simulink model "DC_motor_model"  (R2025b)
settings: Solver=VariableStepAuto  StartTime=0.0  StopTime=10.0  RelTol=1e-3
values from neighbouring files (symbols this model uses):
  K_i = 7.31220718673    [motorbike_cruise_control.mat]
  K_p = 0.333562341287    [motorbike_cruise_control.mat]
  V_max = 11.53    [motorbike_cruise_control.mat]
undefined symbols (not defined in the file or in its folder): K_d, T_s
libraries: slpidlib x1
settings Model: Creator=konstantinos  LastModifiedBy=konstantinos

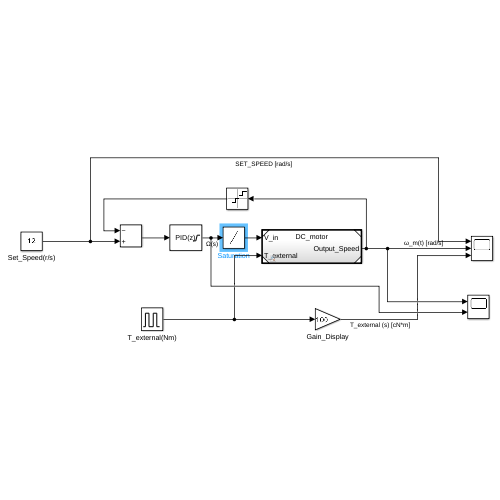
[thumbnail: Simulink's stored preview of the top-level diagram]
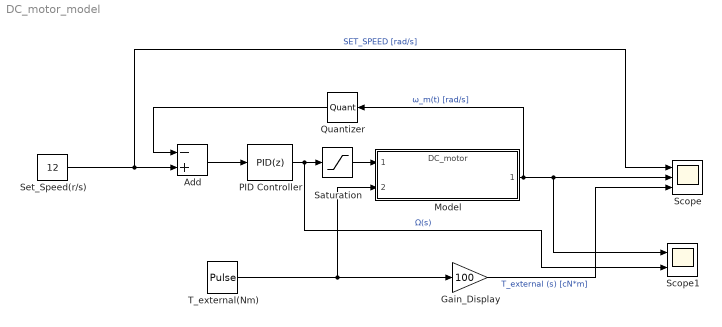
== system DC_motor_model ==
  Add : Sum  Inputs=-+
  Gain_Display : Gain  Gain=100
  Model : ModelReference  ModelNameDialog=DC_motor.slx  SimulationMode=Normal  ModelReferenceVersion=1.4
  PID Controller : slpidlib/PID Controller  Controller=PID  Form=Parallel  TimeDomain=Discrete-time  UseExternalTs=off  SampleTime=T_s  IntegratorMethod=Trapezoidal  FilterMethod=Trapezoidal  ControllerParametersSource=internal  P=K_p  I=K_i  UseKiTs=off  D=K_d  UseExternalDerivativeSource=off  N=100  UseFilter=on  TunerSelectOption=Transfer Function Based (PID Tuner App)  InitialConditionSource=internal  InitialConditionForIntegrator=0  InitialConditionForFilter=0  DifferentiatorICPrevScaledInput=0  ExternalReset=none  TrackingMode=off  Kt=1  LimitOutput=on  SatLimitsSource=internal  UpperSaturationLimit=11.1  LowerSaturationLimit=-11.1  LinearizeAsGain=on  AntiWindupMode=back-calculation  Kb=1  LimitIntegrator=off  UpperIntegratorSaturationLimit=inf  LowerIntegratorSaturationLimit=-inf  POutMin=[]  POutMax=[]  IOutMin=[]  IOutMax=[]  DOutMin=[]  DOutMax=[]  NOutMin=[]  NOutMax=[]  SumOutMin=[]  SumOutMax=[]  SaturationOutMin=[]  SaturationOutMax=[]  PParamMin=[]  PParamMax=[]  IParamMin=[]  IParamMax=[]  DParamMin=[]  DParamMax=[]  NParamMin=[]  NParamMax=[]  KbParamMin=[]  KbParamMax=[]  KtParamMin=[]  KtParamMax=[]  KbOutMin=[]  KbOutMax=[]  KtOutMin=[]  KtOutMax=[]  IntegratorOutMin=[]  IntegratorOutMax=[]  FilterOutMin=[]  FilterOutMax=[]  SumI1OutMin=[]  SumI1OutMax=[]  SumI2OutMin=[]  SumI2OutMax=[]  SumI3OutMin=[]  SumI3OutMax=[]  SumI4OutMin=[]  SumI4OutMax=[]  SumDOutMin=[]  SumDOutMax=[]  DifferentiatorOutMin=[]  DifferentiatorOutMax=[]  FilterDiffOutCoefMin=[]  FilterDiffOutCoefMax=[]  ReciprocalOutMin=[]  ReciprocalOutMax=[]  SumDenOutMin=[]  SumDenOutMax=[]  SumNumOutMin=[]  SumNumOutMax=[]  DivideOutMin=[]  DivideOutMax=[]  UdiffTsProdOutMin=[]  UdiffTsProdOutMax=[]  NTsProdOutMin=[]  NTsProdOutMax=[]  UintegralTsProdOutMin=[]  UintegralTsProdOutMax=[]  UngainTsProdOutMin=[]  UngainTsProdOutMax=[]  ClampingZeroOutDataTypeStr=Inherit: Inherit via back propagation  ClampingZeroOutMin=[]  ClampingZeroOutMax=[]  FilterDenConstantOutDataTypeStr=Inherit: Inherit via back propagation  FilterDenConstantOutMin=[]  FilterDenConstantOutMax=[]  PCopyOutDataTypeStr=Inherit: Inherit via back propagation  PCopyOutMin=[]  PCopyOutMax=[]  NCopyOutDataTypeStr=Inherit: Inherit via back propagation  NCopyOutMin=[]  NCopyOutMax=[]  IntegratorContinuousStateAttributes=''  IntegratorStateMustResolveToSignalObject=off  IntegratorRTWStateStorageClass=Auto  FilterContinuousStateAttributes=''  FilterStateMustResolveToSignalObject=off  FilterRTWStateStorageClass=Auto  ParallelPVariant=InternalParameters  IdealPVariant=Disabled  IVariant=InternalParameters  DVariant=InternalParameters  IntegratorVariant=Discrete  SatVariant=Enabled  AWVariant=BackCalculation  PCopyVariant=Disabled  TRVariant=Disabled  FdbkBlocksVariant=Feedback  IdealPFdbkVariant=Passthrough  SatFdbkVariant=Enabled  DerivativeFilterVariant=TrapezoidalFilter  NVariant=InternalParameters  NCopyVariant=InternalParameters  FilterICVariant=InternalICsFilter  IntegratorICVariant=InternalICs  ExternalResetVariant=Disabled  TRSumVariant=Passthrough  SumFdbkVariant=Enabled  SumVariant=Sum_PID  TsampFilterVariant=InternalTs  TsampNgainVariant=Passthrough  TsampIntegralVariant=Disabled_SignalSpec  ExternalSaturationOutDataTypeStr=Inherit: Same as second input  DerivativeSourceVariant=ErrorSignal  PreIntVariant=InternalPreInt
  Quantizer : Quantizer  QuantizationInterval=2*pi/1200
  Saturation : Saturate  UpperLimit=V_max  LowerLimit=-V_max
  Scope : Scope  NumInputPorts=3
      settings: ActiveDisplayYMinimum=-9.4133876300961674  ActiveDisplayYMaximum=29.145633273501279
  Scope1 : Scope  NumInputPorts=2
      settings: ActiveDisplayYMinimum=-5.6083033873767807  ActiveDisplayYMaximum=27.783538480087149
  Set_Speed(r/s) : Constant  Value=12
  T_external(Nm) : DiscretePulseGenerator  PulseType=Time based  Amplitude=0.01  Period=4  PulseWidth=25  PhaseDelay=1
  wires:
  Add/1 -> PID Controller/1
  Model/1 -> Quantizer/1, Scope1/1, Scope/2  "ω_m(t) [rad/s]"
  PID Controller/1 -> Scope1/2, Saturation/1  "Ω(s)"
  Set_Speed(r/s)/1 -> Scope/1, Add/2  "SET_SPEED [rad/s]"
  T_external(Nm)/1 -> Model/2, Gain_Display/1
  Gain_Display/1 -> Scope/3  "T_external (s) [cN*m]"
  Quantizer/1 -> Add/1
  Saturation/1 -> Model/1
